simulink model "Dual_Clutch_Trans_SDO"  (R2025a)
settings: Solver=ode1  StartTime=0.0  StopTime=15  MaxStep=0.1  RelTol=1e-3  EnableMultiTasking=on
PreLoadFcn:
  | load UrbanCycle1;
  | load UrbanCycle2;
  | load UrbanCycle3;
  | load UrbanCycle4;
  | load UrbanCycle5;
  | load UrbanCycle6;
  | load UrbanCycle7;
  | load UrbanCycle8;
  | Shift_Gear_Delay = 50;
  | Ratio_Time_Const = 0.1;
  | Drive_Cycle_Num = 7;
  | load RefRPMData;
PostLoadFcn:
  | warning off Simulink:SampleTime:TsPropEnabOutputsChangeNotAligned;
  | warning off Simulink:blocks:MatchingFromNotFound
  | warning off Simulink:blocks:MatchingGotoNotFound
  | warning off Simulink:Engine:OutputNotConnected
  | warning off Simulink:Engine:LineWithoutDst
  | warning off Simulink:Engine:UINotUpdatedDuringRapidAccelSim
  | warning off Simulink:Commands:SetParamLinkChangeWarn
  | warning off Simulink:Engine:SaveWithParameterizedLinks_Warning
undefined symbols (not defined in the file or in its folder): DCT_Param, Downshift_Speeds, sigbuilder_block, Upshift_Speeds
libraries: fl_lib x5, nesl_utility x4, sdl_lib x2, simulink x2, DCT_Vehicle_Dynamics_Lib x2, Engine_Lib x1, slpidlib x1
(part 2 of 2)

== system Dual_Clutch_Trans_SDO/Transmission Controller/Gear shift demands/Create pulse if next gear number changes and CL2 is not engaged ==
  ~E : Inport
  nG : Inport  Port=2
  0.5s delay : Delay  DelayLength=DCT_Param.Dog_Clutches.Pulse_Length  SampleTime=0.01
  Abs : Abs
  Create a 1/2s pulse if not engaged and the next gear number changes : Product  InputSameDT=on  SaturateOnIntegerOverflow=on  OutDataTypeStr=Inherit: Same as first input
  Rate Transition : RateTransition  OutPortSampleTime=0.01
  Rate Transition1 : RateTransition  OutPortSampleTime=0.01
  Sum2 : Sum  Inputs=|+-  InputSameDT=on  SaturateOnIntegerOverflow=on  OutDataTypeStr=Inherit: Same as first input
  "[0,1]" : Saturate  UpperLimit=1  LowerLimit=0
  Pulse : Outport  VectorParamsAs1DForOutWhenUnconnected=off
  wires:
  ~E/1 -> Create a 1/2s pulse if not engaged and the next gear number changes/2
  Create a 1/2s pulse if not engaged and the next gear number changes/1 -> Pulse/1
  "[0,1]"/1 -> Rate Transition/1
  Abs/1 -> "[0,1]"/1
  Sum2/1 -> Abs/1
  0.5s delay/1 -> Sum2/1
  nG/1 -> Rate Transition1/1
  Rate Transition/1 -> Create a 1/2s pulse if not engaged and the next gear number changes/1
  Rate Transition1/1 -> Sum2/2, 0.5s delay/1

== system Dual_Clutch_Trans_SDO/Transmission Controller/Shift state/Chart/calc ==
  note: Determine if next gear will be
      | higher or lower than current gear
  gear : Inport
  pedal : Inport  Port=2
  speed : Inport  Port=3
  f : TriggerPort  TriggerType=function-call  VariantControl=Variant
      settings: CopyFcn=Stateflow.SLINSF.SimulinkMan.removeBlockPreDeleteFcn  PreDeleteFcn=Stateflow.SLINSF.SimulinkMan.unsafePredeleteFcn
  Add1 : Sum  Inputs=+-
  Add3 : Sum  Inputs=+-
  Add4 : Sum  Inputs=+-
  Calculate Downshift Threshold : Lookup2D  RowIndex=DCT_Param.Shift_Map.Pedal_Positions  ColumnIndex=[2,3,4,5,6]  Table=DCT_Param.Shift_Map.Downshift_Speeds  LookUpMeth=Interpolation-Use End Values  SaturateOnIntegerOverflow=off  InputSameDT=off
  Calculate Upshift Threshold : Lookup2D  RowIndex=Pedal_Positions  ColumnIndex=[1,2,3,4,5]  Table=Upshift_Speeds  LookUpMeth=Interpolation-Use End Values  SaturateOnIntegerOverflow=off  InputSameDT=off
  SpdThr : Outport  VectorParamsAs1DForOutWhenUnconnected=off
  wires:
  Add4/1 -> SpdThr/1
  Add3/1 -> Add4/2
  Add1/1 -> Add4/1
  speed/1 -> Add3/1, Add1/2
  Calculate Upshift Threshold/1 -> Add1/1
  Calculate Downshift Threshold/1 -> Add3/2
  gear/1 -> Calculate Downshift Threshold/2, Calculate Upshift Threshold/2
  pedal/1 -> Calculate Downshift Threshold/1, Calculate Upshift Threshold/1

== system Dual_Clutch_Trans_SDO/Transmission Controller/Shift state/Chart/calc_down ==
  gear : Inport
  pedal : Inport  Port=2
  f : TriggerPort  TriggerType=function-call  VariantControl=Variant
      settings: CopyFcn=Stateflow.SLINSF.SimulinkMan.removeBlockPreDeleteFcn  PreDeleteFcn=Stateflow.SLINSF.SimulinkMan.unsafePredeleteFcn
  Calculate Downshift Threshold : Lookup2D  RowIndex=Pedal_Positions  ColumnIndex=[2,3,4,5,6]  Table=Downshift_Speeds  LookUpMeth=Interpolation-Use End Values  SaturateOnIntegerOverflow=off  InputSameDT=off
  down_th : Outport  VectorParamsAs1DForOutWhenUnconnected=off
  wires:
  pedal/1 -> Calculate Downshift Threshold/1
  gear/1 -> Calculate Downshift Threshold/2
  Calculate Downshift Threshold/1 -> down_th/1

== system Dual_Clutch_Trans_SDO/Transmission Controller/Shift state/Chart/calc_up ==
  gear : Inport
  pedal : Inport  Port=2
  f : TriggerPort  TriggerType=function-call  VariantControl=Variant
      settings: CopyFcn=Stateflow.SLINSF.SimulinkMan.removeBlockPreDeleteFcn  PreDeleteFcn=Stateflow.SLINSF.SimulinkMan.unsafePredeleteFcn
  Calculate Upshift Threshold : Lookup2D  RowIndex=Pedal_Positions  ColumnIndex=[1,2,3,4,5]  Table=Upshift_Speeds  LookUpMeth=Interpolation-Use End Values  SaturateOnIntegerOverflow=off  InputSameDT=off
  up_th : Outport  VectorParamsAs1DForOutWhenUnconnected=off
  wires:
  gear/1 -> Calculate Upshift Threshold/2
  pedal/1 -> Calculate Upshift Threshold/1
  Calculate Upshift Threshold/1 -> up_th/1

== system Dual_Clutch_Trans_SDO/Transmission Controller/Shift state/Enable Clutch ==
  nG : Inport
  0.5s delay : Delay  DelayLength=DCT_Param.Dog_Clutches.Pulse_Length  SampleTime=0.01
  Relational Operator : RelationalOperator  Operator===  OutDataTypeStr=boolean  InputSameDT=off
  Zero-Order Hold : ZeroOrderHold  SampleTime=DCT_Param.Dog_Clutches.Pulse_Length*0.01
  Clutch : Outport  VectorParamsAs1DForOutWhenUnconnected=off
  wires:
  0.5s delay/1 -> Relational Operator/1
  Zero-Order Hold/1 -> 0.5s delay/1, Relational Operator/2
  nG/1 -> Zero-Order Hold/1
  Relational Operator/1 -> Clutch/1

== system Dual_Clutch_Trans_SDO/Transmission Controller/Shift state/Permit Clutch Change ==
  C1_Cmd : Inport
  C2_Cmd : Inport  Port=2
  Enable : EnablePort
  C1 : Outport  VectorParamsAs1DForOutWhenUnconnected=off
  C2 : Outport  Port=2  VectorParamsAs1DForOutWhenUnconnected=off
  wires:
  C1_Cmd/1 -> C1/1
  C2_Cmd/1 -> C2/1

== system Dual_Clutch_Trans_SDO/Abstracted/Gears/Ratio Selection/Lag Filter with IC ==
  In : Inport
  Gain : Gain  Gain=1/b
  Integrator : Integrator  InitialCondition=x_initial*b
  Sum : Sum  Inputs=|+-  InputSameDT=on  SaturateOnIntegerOverflow=on  OutDataTypeStr=Inherit: Same as first input
  Out : Outport  VectorParamsAs1DForOutWhenUnconnected=off
  wires:
  Gain/1 -> Out/1, Sum/2
  Integrator/1 -> Gain/1
  In/1 -> Sum/1
  Sum/1 -> Integrator/1

== system Dual_Clutch_Trans_SDO/Transmission Controller/Clutch Pressure Control/Clutch 1 Pressure Launch/Inverse clutch model ==
  Trq : Inport
  Trq2P : Gain  Gain=1/(N*r_eff*mu*A)  SaturateOnIntegerOverflow=on  OutDataTypeStr=Inherit: Same as input  ParamDataTypeStr=Inherit: Same as input
  P : Outport  VectorParamsAs1DForOutWhenUnconnected=off
  wires:
  Trq2P/1 -> P/1
  Trq/1 -> Trq2P/1

== stateflow chart Dual_Clutch_Trans_SDO/Transmission Controller/Shift state/Chart ==
  settings: sampleTime=0.01
  state GearState [parallel]
    settings: executionOrder=1
    state G1
      en: GearState=1;
      en:C1=1;C2=0;
      NGsf=2;
    state G3
      en: GearState=3;
      du:[SpdThr]=calc(3,pedal,speed);
      (history)
      state NGlow
        en: NGsf=2;
      state NGhigh
        en: NGsf=4;
      (default) -> GearState.G3.NGlow
      GearState.G3.NGlow -> GearState.G3.NGhigh : [SpdThr<0 &&...
          | GearState==3]
      GearState.G3.NGhigh -> GearState.G3.NGlow : [SpdThr>=0 &&...
          | GearState==3]
    state G2
      en: GearState=2;
      du:[SpdThr]=calc(2,pedal,speed);
      (history)
      state NGlow
        en: NGsf=1;
      state NGhigh
        en: NGsf=3;
      (default) -> GearState.G2.NGlow
      GearState.G2.NGlow -> GearState.G2.NGhigh : [SpdThr<0 &&...
          |  GearState==2]
      GearState.G2.NGhigh -> GearState.G2.NGlow : [SpdThr>=0 &&...
          |  GearState==2]
    state Launch
      en: GearState=0.5;
      en:C1=0;C2=0;
      NGsf=1;
    state G5
      en:GearState=5;
      du:[SpdThr]=calc(5,pedal,speed);
      (history)
      state NGlow
        en: NGsf=4;
      state NGhigh
        en: NGsf=6;
      (default) -> GearState.G5.NGlow
      GearState.G5.NGlow -> GearState.G5.NGhigh : [SpdThr<0 &&...
          | GearState==5]
      GearState.G5.NGhigh -> GearState.G5.NGlow : [SpdThr>=0 &&...
          | GearState==5]
    state G6
      en:GearState=6;
      NGsf=5;
    state G4
      en:GearState=4;
      du:[SpdThr]=calc(4,pedal,speed);
      (history)
      state NGlow
        en: NGsf=3;
      state NGhigh
        en: NGsf=5;
      (default) -> GearState.G4.NGlow
      GearState.G4.NGlow -> GearState.G4.NGhigh : [SpdThr<0 &&...
          | GearState==4]
      GearState.G4.NGhigh -> GearState.G4.NGlow : [SpdThr>=0 &&...
          | GearState==4]
    G1 -> G2 [order 1] : Up
    Launch -> G1 : [abs(S1)<10 && RPM>850]
        | {clutchControl=1;}
    G2 -> G3 [order 1] : Up
    G3 -> G2 [order 2] : Down
    G1 -> Launch [order 2] : [RPM<800]
        | {clutchControl=-1;}
    G2 -> G1 [order 2] : Down
    (default) -> Launch
    G3 -> G4 [order 1] : Up
    G4 -> G3 [order 2] : Down
    G4 -> G5 [order 1] : Up
    G5 -> G6 [order 1] : Up
    G6 -> G5 : Down
    G5 -> G4 [order 2] : Down
  state SelectionState [parallel]
    du:[up_th]=calc_up(GearState,pedal);
    du:[down_th]=calc_down(GearState,pedal);
    settings: executionOrder=2
    state SteadyState
      en:clutchControl=0;
    state preDownShifting
    state preUpShifting
    state UpShifting
      en: GearState=GearState+0.5;
      en:[C1,C2] = clutchstates...
      (GearState,clutchControl)
    state DownShifting
      en: GearState=GearState-0.5;
      en:[C1,C2] = clutchstates...
      (GearState,clutchControl)
    (default) -> SteadyState
    SteadyState -> (junction 62) [order 1] : [speed < down_th && ...
        | GearState >1]
        | {clutchControl=-1;}
    SteadyState -> (junction 128) [order 2] : [speed > up_th &&...
        | GearState <=5 && ...
        | floor(GearState) == GearState]
        | {clutchControl=1;}
    (junction 62) -> preDownShifting
    (junction 128) -> preUpShifting
    (junction 168) -> SteadyState
    (junction 23) -> SteadyState
    (junction 161) -> SteadyState
    preDownShifting -> (junction 168) [order 2] : [speed >= down_th]
    preUpShifting -> (junction 161) [order 2] : [speed <= up_th]
    preUpShifting -> UpShifting [order 1] : after(0.5,sec)
        | [speed>up_th]
    preDownShifting -> DownShifting [order 1] : after(0.5,sec)
        | [speed < down_th-2]
    DownShifting -> (junction 23) : [shiftComplete ==1]
        | {GearState.Down;}
    UpShifting -> (junction 23) : [shiftComplete==1]
        | {GearState.Up;}
  state up_th = calc_up(gear,pedal) [function]
  state down_th = calc_down(gear,pedal) [function]
  state SpdThr = calc(gear,pedal,speed) [function]
  data: gear function_input; pedal function_input; up_th function_output; gear function_input; pedal function_input; down_th function_output; gear function_input; pedal function_input; SpdThr function_output; speed function_input; gear function_input double; updown function_input double; cl1 function_output double; cl2 function_output double; GearState output double; S1 input; shiftComplete input; speed input; pedal input; up_th output double; down_th output double; RPM input; NGsf output double; C1 output double; C2 output double; clutchControl local double; SpdThr local double
  events: Up local EITHER_EDGE_EVENT; Down local EITHER_EDGE_EVENT
  function [cl1,cl2] = clutchstates(gear,updown):
    | function [cl1,cl2] = clutchstates(gear,updown) 
    | if (((gear==1.5)||(gear==3.5)||(gear==5.5))&&(updown==1) || ((gear==2.5)||(gear==4.5))&&(updown==-1))
    |     cl1 = 0;
    |     cl2 = 1;
    | else%if((gear==1.5)||(gear==3.5))&&(updown==-1) || ((gear==2.5)||(gear==4.5))&&(updown==1)
    | 	cl1 = 1;
    |     cl2 = 0;
    | end
